simulink model "asbCubeSatEnvironment"  (R2025b)
settings: configuration reference "CubeSatConfigSet" (kept outside this file)
undefined symbols (not defined in the file): CubeSatTimeStep
libraries: asbCubeSatEnvironmentLib x1
settings Model: DataDictionary=asbCubeSatArchInterfaceData.sldd  Creator=The MathWorks, Inc.  LastModifiedBy=The MathWorks, Inc.
settings ConfigSetRef: SourceName=CubeSatConfigSet

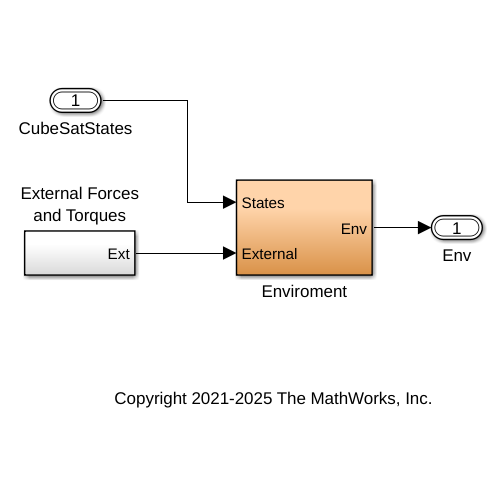
[thumbnail: Simulink's stored preview of the top-level diagram]
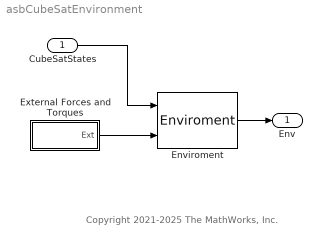
== system asbCubeSatEnvironment ==
  note: Copyright 2021-2025 The MathWorks, Inc.
  CubeSatStates : Inport  OutDataTypeStr=Bus: StatesOutBus
  Enviroment : asbCubeSatEnvironmentLib/Enviroment  SystemSampleTime=-1  VariantActivationTime=update diagram  EmptyChoice=off  PassThrough=off  PassThroughVariantControl=(default)  EmptyChoiceVariantControl=(default)  AllowFlexibleInterface=on  Latency=0  AutoFrameSizeCalculation=off
  "External Forces and Torques " : Subsystem
  Env : Outport  OutDataTypeStr=Bus: EnvBus
  wires:
  "External Forces and Torques "/1(Ext) -> Enviroment/2
  Enviroment/1 -> Env/1
  CubeSatStates/1 -> Enviroment/1

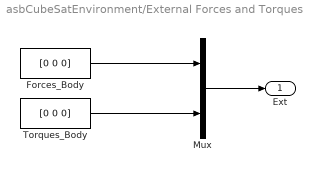
== system asbCubeSatEnvironment/External Forces and Torques  ==
  Forces_Body : Constant  Value=[0 0 0]  SampleTime=CubeSatTimeStep
  Mux : Mux  Inputs=2
  Torques_Body : Constant  Value=[0 0 0]  SampleTime=CubeSatTimeStep
  Ext : Outport  VectorParamsAs1DForOutWhenUnconnected=off
  wires:
  Forces_Body/1 -> Mux/1
  Torques_Body/1 -> Mux/2
  Mux/1 -> Ext/1
